simulink model "TPWMMems2023"  (R2023a)
settings: Solver=ode4  StartTime=0.0  StopTime=1  FixedStep=0.01  RelTol=1e-3
libraries: AFCToolbox x8
settings Model: Creator=Administrator  LastModifiedBy=zqhkd
settings OptimizationCC: DefaultParameterBehavior=Inlined  EnhancedBackFolding=on  PassReuseOutputArgsAs=Individual arguments  ZeroExternalMemoryAtStartup=off  ZeroInternalMemoryAtStartup=off  OptimizeBlockOrder=speed  DifferentSizesBufferReuse=on  OptimizationCustomize=off  EfficientTunableParamExpr=on
settings DebuggingCC: ParameterPrecisionLossMsg=none  ParameterTunabilityLossMsg=error
settings HardwareCC: ProdBitPerInt=16  ProdBitPerPointer=16  ProdBitPerSizeT=16  ProdBitPerPtrDiffT=16  ProdLargestAtomicFloat=None  ProdWordSize=16  ProdHWDeviceType=STMicroelectronics->ST10/Super10
settings SFSimCC: MATLABDynamicMemAlloc=off
settings RTWCC: Description=Embedded Coder  SystemTargetFile=AFCHawk.tlc  GenCodeOnly=on  TemplateMakefile=ert_default_tmf
settings CodeAppCC: ForceParamTrailComments=on  IgnoreCustomStorageClasses=off  OperatorAnnotations=on  SimulinkDataObjDesc=on  SFDataObjDesc=on  InsertBlockDesc=on
settings STFCustomTargetCC: MultiwordLength=256  ModelReferenceCompliant=off  ConcurrentExecutionCompliant=off  CombineOutputUpdateFcns=on  ERTCustomFileBanners=on  SupportContinuousTime=off  SupportNonInlinedSFcns=off  RemoveResetFunc=on  MATLABClassNameForMDSCustomization=Simulink.SoftwareTarget.ERTCustomization  GRTInterface=off  UseToolchainInfoCompliant=off  SystemTargetFile=AFCHawk.tlc
settings ERTTargetCC: TargetLangStandard=C99 (ISO)  ModelReferenceCompliant=off  ParMdlRefBuildCompliant=off  CompOptLevelCompliant=off  ConcurrentExecutionCompliant=off  ModelStepFunctionPrototypeControlCompliant=off  CPPClassGenCompliant=off  UseToolchainInfoCompliant=off  InlinedParameterPlacement=NonHierarchical  ERTCustomFileTemplate=example_file_process.tlc
settings ConfigComp: CovBoundaryAbsTol=1.0e-5

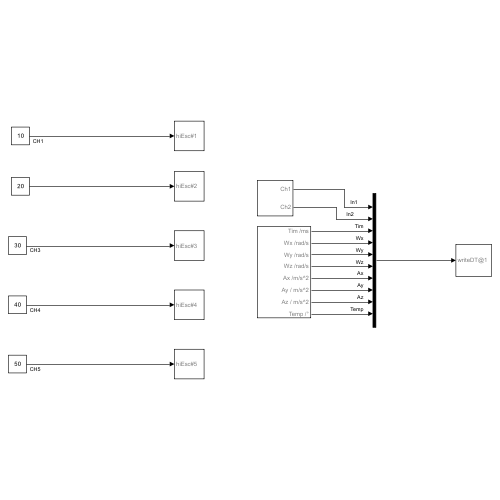
[thumbnail: Simulink's stored preview of the top-level diagram]
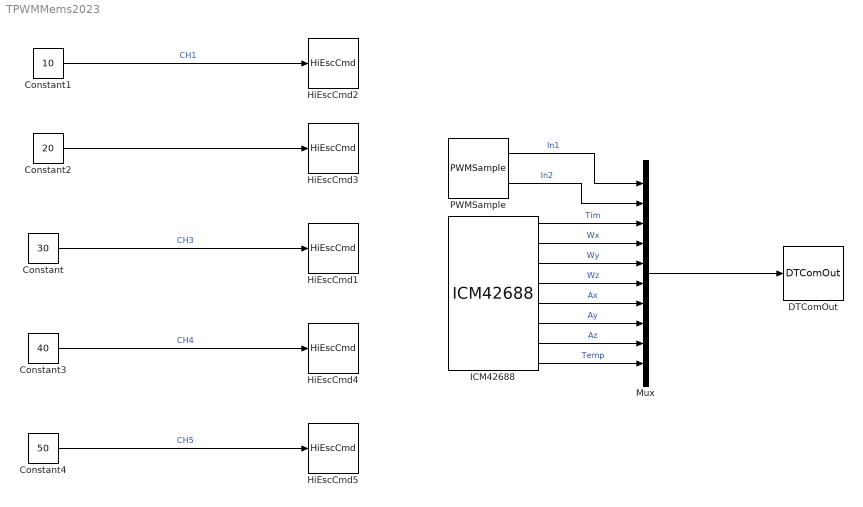
== system TPWMMems2023 ==
  Constant : Constant  Value=30
  Constant1 : Constant  Value=10
  Constant2 : Constant  Value=20
  Constant3 : Constant  Value=40
  Constant4 : Constant  Value=50
  DTComOut : AFCToolbox/DeviceModule/DTComOut  Priority=8  g_frameType=1  g_outFreq=1  g_comPort=0  g_instName=0  g_id=0
      settings: SourceProductName=AFCToolbox
  HiEscCmd1 : AFCToolbox/DeviceModule/HiEscCmd  Priority=6  g_chanelNo=3  g_minPW=0  g_maxPW=100  g_comPort=6  g_instName=0  g_id=0
      settings: SourceProductName=AFCToolbox
  HiEscCmd2 : AFCToolbox/DeviceModule/HiEscCmd  Priority=6  g_chanelNo=1  g_minPW=0  g_maxPW=100  g_comPort=6  g_instName=0  g_id=0
      settings: SourceProductName=AFCToolbox
  HiEscCmd3 : AFCToolbox/DeviceModule/HiEscCmd  Priority=6  g_chanelNo=2  g_minPW=0  g_maxPW=100  g_comPort=6  g_instName=0  g_id=0
      settings: SourceProductName=AFCToolbox
  HiEscCmd4 : AFCToolbox/DeviceModule/HiEscCmd  Priority=6  g_chanelNo=4  g_minPW=0  g_maxPW=100  g_comPort=6  g_instName=0  g_id=0
      settings: SourceProductName=AFCToolbox
  HiEscCmd5 : AFCToolbox/DeviceModule/HiEscCmd  Priority=6  g_chanelNo=5  g_minPW=0  g_maxPW=100  g_comPort=6  g_instName=0  g_id=0
      settings: SourceProductName=AFCToolbox
  ICM42688 : AFCToolbox/DeviceModule/ICM42688  Priority=0  g_sampleTime=0.01  g_comPort=6  g_instName=0  g_id=0
      settings: SourceProductName=AFCToolbox
  Mux : Mux  Inputs=10
  PWMSample : AFCToolbox/DeviceModule/PWMSample  Priority=1  g_sampleTime=0.01  g_comPort=6  g_instName=0  g_id=0
      settings: SourceProductName=AFCToolbox
  wires:
  PWMSample/1 -> Mux/1  "In1"
  PWMSample/2 -> Mux/2  "In2"
  Mux/1 -> DTComOut/1
  Constant/1 -> HiEscCmd1/1  "CH3"
  Constant1/1 -> HiEscCmd2/1  "CH1"
  Constant2/1 -> HiEscCmd3/1
  Constant3/1 -> HiEscCmd4/1  "CH4"
  Constant4/1 -> HiEscCmd5/1  "CH5"
  ICM42688/1 -> Mux/3  "Tim"
  ICM42688/2 -> Mux/4  "Wx"
  ICM42688/3 -> Mux/5  "Wy"
  ICM42688/4 -> Mux/6  "Wz"
  ICM42688/5 -> Mux/7  "Ax"
  ICM42688/6 -> Mux/8  "Ay"
  ICM42688/7 -> Mux/9  "Az"
  ICM42688/8 -> Mux/10  "Temp"
